simulink model "TestMotors"  (R2022b)
settings: Solver=FixedStepAuto  StartTime=0.0  StopTime=10.0  RelTol=1e-3  EnableMultiTasking=on
libraries: arduinolib x6, simulink x2
settings Model: ExtModeTrigDuration=2  Creator=miriamfreiriasanjuan  LastModifiedBy=miriamfreiriasanjuan
settings OptimizationCC: EnhancedBackFolding=on  PassReuseOutputArgsAs=Individual arguments  ZeroExternalMemoryAtStartup=off  ZeroInternalMemoryAtStartup=off  MaxStackSize=64  OptimizeBlockOrder=speed  DifferentSizesBufferReuse=on  OptimizationCustomize=off  EfficientTunableParamExpr=on
settings DebuggingCC: ParameterTunabilityLossMsg=error
settings HardwareCC: ProdBitPerInt=16  ProdBitPerPointer=16  ProdBitPerSizeT=16  ProdBitPerPtrDiffT=16  ProdLargestAtomicFloat=None  ProdWordSize=8  ProdHWDeviceType=Atmel->AVR
settings SFSimCC: MATLABDynamicMemAlloc=off
settings RTWCC: Description=Embedded Coder  SystemTargetFile=ert.tlc  HardwareBoard=Arduino Mega 2560  TLCOptions=-aInlineSetEventsForThisBaseRateFcn=TLC_FALSE -aSuppressMultiTaskScheduler=TLC_FALSE -aRateBasedStepFcn=1  TemplateMakefile=ert_default_tmf  Toolchain=Arduino AVR  BuildConfiguration=Faster Runs
settings CodeAppCC: ForceParamTrailComments=on  IgnoreCustomStorageClasses=off  OperatorAnnotations=on  SimulinkDataObjDesc=on  SFDataObjDesc=on  InsertBlockDesc=on
settings ERTTargetCC: SupportContinuousTime=on  SupportVariableSizeSignals=on  ExtModeTransport=3  ExtModeStaticAlloc=on  ExtModeAutomaticAllocSize=off  ExtModeStaticAllocSize=2048  ExtModeMexFile=ext_xcp  ExtModeIntrfLevel=Level2 - Open

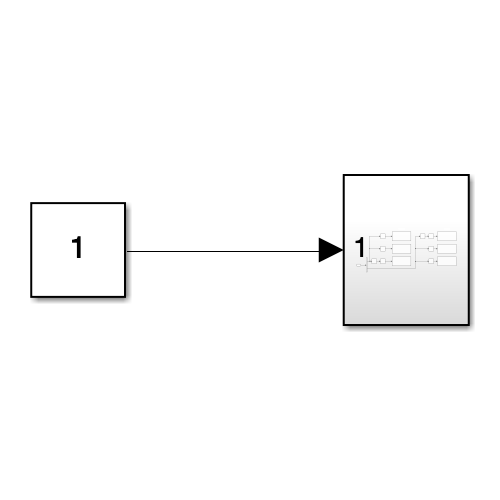
[thumbnail: Simulink's stored preview of the top-level diagram]
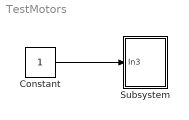
== system TestMotors ==
  Constant : Constant
  Subsystem : Subsystem
  wires:
  Constant/1 -> Subsystem/1(In3)

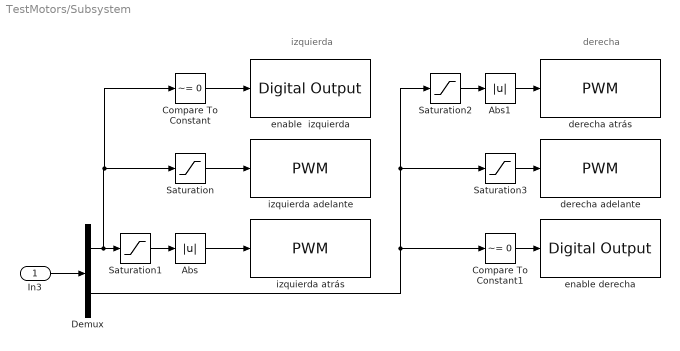
== system TestMotors/Subsystem ==
  note: derecha
  note: izquierda
  In3 : Inport
  Abs : Abs  SaturateOnIntegerOverflow=off
  Abs1 : Abs  SaturateOnIntegerOverflow=off
  Compare To Constant : simulink/Logic and Bit Operations/Compare To Constant  relop=~=  const=0  OutDataTypeStr=boolean
  Compare To Constant1 : simulink/Logic and Bit Operations/Compare To Constant  relop=~=  const=0  OutDataTypeStr=boolean
  Demux : Demux  Outputs=2
  Saturation : Saturate  UpperLimit=255  LowerLimit=0
  Saturation1 : Saturate  UpperLimit=0  LowerLimit=-255
  Saturation2 : Saturate  UpperLimit=0  LowerLimit=-255
  Saturation3 : Saturate  UpperLimit=255  LowerLimit=0
  derecha adelante : arduinolib/PWM  pinNumber=5  frequencyType=Default  desiredFrequency=490.2  achievableFrequency=490.2
  derecha atrás : arduinolib/PWM  pinNumber=5  frequencyType=Default  desiredFrequency=490.2  achievableFrequency=490.2
  enable  izquierda : arduinolib/Digital Output  pinNumber=9  Direction=output  blockPlatform=arduino
  enable derecha : arduinolib/Digital Output  pinNumber=9  Direction=output  blockPlatform=arduino
  izquierda adelante : arduinolib/PWM  pinNumber=5  frequencyType=Default  desiredFrequency=490.2  achievableFrequency=490.2
  izquierda atrás : arduinolib/PWM  pinNumber=5  frequencyType=Default  desiredFrequency=490.2  achievableFrequency=490.2
  wires:
  Saturation3/1 -> derecha adelante/1
  Abs/1 -> izquierda atrás/1
  Demux/1 -> Compare To Constant/1, Saturation/1, Saturation1/1
  Compare To Constant1/1 -> enable derecha/1
  Saturation2/1 -> Abs1/1
  Saturation1/1 -> Abs/1
  In3/1 -> Demux/1
  Compare To Constant/1 -> enable  izquierda/1
  Saturation/1 -> izquierda adelante/1
  Demux/2 -> Compare To Constant1/1, Saturation3/1, Saturation2/1
  Abs1/1 -> derecha atrás/1
